simulink model "sf_pole_vault"  (R2025b)
settings: Solver=VariableStepAuto  StartTime=0.0  StopTime=4  MaxStep=.0002  RelTol=1e-3  EnableMultiTasking=on
PreLoadFcn:
  | Params.angle=30;
  | Params.x0=10;
  | Params.y0=3;
  | Params.K=300;
  | Params.mass=100;
  | Params.Pole=4;
  | ang=Params.angle;
  | theta0=ang*pi/180;
  | ltheta0=(Params.x0*sin(theta0)+Params.y0*cos(theta0))/4;
  | r0=Params.y0*sin(theta0)-Params.x0*cos(theta0);
libraries: simulink_extras x3, simulink x1
settings Model: PauseTimes=1.31  Creator=The MathWorks, Inc.  LastModifiedBy=The MathWorks, Inc.
settings SolverCC: AlgebraicLoopSolver=TrustRegion  MaxZcPerStep=1.0
settings DataIOCC: ReturnWorkspaceOutputs=off
settings OptimizationCC: ReuseModelBlockBuffer=off  LifeSpan=inf
settings DebuggingCC: UnconnectedInputMsg=warning  UnconnectedOutputMsg=warning  UnconnectedLineMsg=warning  SFUnexpectedBacktrackingDiag=warning  SFNoUnconditionalDefaultTransitionDiag=warning  SFExecutionAtInitializationDiag=none  ArithmeticOperatorsInVariantConditions=warning
settings ModelReferenceCC: EnableRefExpFcnMdlSchedulingChecks=on
settings SFSimCC: SimUseLocalCustomCode=off  CustomCodeUndefinedFunction=UseInterfaceOnly
settings RTWCC: RTWUseLocalCustomCode=off  GPUComputeCapability=3.5  DLArmComputeVersion=19.05
settings CodeAppCC: StateflowObjectComments=on
settings GRTTargetCC: TargetLangStandard=C89/C90 (ANSI)
settings ConfigComp: CovScope=ReferencedModels  CovIncludeTopModel=off  CovMetricSettings=dw  CovSaveCumulativeToWorkspaceVar=on  CovSaveSingleToWorkspaceVar=on  CovExternalEMLEnable=off

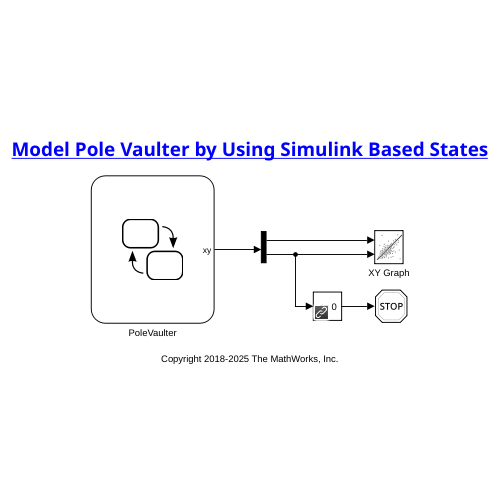
[thumbnail: Simulink's stored preview of the top-level diagram]
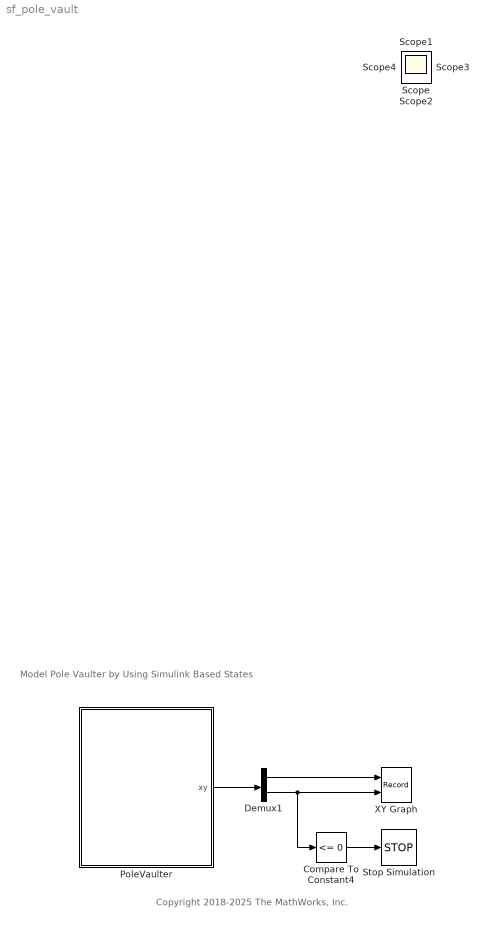
== system sf_pole_vault ==
  note: Copyright 2018-2025 The MathWorks, Inc.
  note: Model Pole Vaulter by Using Simulink Based States
  Compare To Constant4 : simulink/Logic and Bit Operations/Compare To Constant  relop=<=  const=0  OutDataTypeStr=boolean
  Demux1 : Demux  Outputs=2
  PoleVaulter : Stateflow chart  TreatAsAtomicUnit=on
  Stop Simulation : Stop
  XY Graph : Record  NumPorts=2.0  FileSettingsInternal="{\"entries\":[{\"content\":{\"excelSettings\":{\"content\":{},\"type\":\"Streamout.ExcelSettings\"},\"parquetSettings\":{\"content\":{},\"type\":\"Streamout.ParquetSettings\"}},\"type\":\"Streamout.FileSettingStorage\",\"uuid\":\"\"}],\"packageUris\":[\"http:\\/\\/schema.mathworks.com\\/mf0\\/streamout_blocks\\/R2020a\"],\"version\":\"1.0\"}"  FrameSettings=[0, 0]  Layout=[1 1]  SignalsInternal="{\"entries\":[{\"content\":{\"signals\":[{\"content\":{\"blockPath\":[],\"dimensions\":[1],\"domain\":\"\",\"lineColor\":\"#a2142f\",\"plots\":[ 1 ],\"port\":1,\"signalID\":1,\"signalName\":\"XY Graph:1\"},\"type\":\"RecordBlkView.Signal\",\"uuid\":\"\"},{\"content\":{\"blockPath\":[],\"dimensions\":[1],\"domain\":\"\",\"lineColor\":\"#139fff\",\"plots\":[ 1 ],\"port\":2,\"signalID\":2,\"signalName\":\"XY Graph:2\"},\"type\":\"RecordBlkView.Signal\",\"uuid\":\"\"}]},\"type\":\"RecordBlkView.InputSignals\",\"uuid\":\"\"}],\"packageUris\":[\"http:\\/\\/schema.mathworks.com\\/mf0\\/streamout_blocks\\/R2020a\"],\"version\":\"1.0\"}"  VisualizationBindings="{\"xyplotplugin\":{\"info\":[{\"series\":[{\"bindingParametersList\":[{\"parameter\":\"X-Axis\",\"signalID\":1,\"signalName\":\"XY Graph:1\"},{\"parameter\":\"Y-Axis\",\"signalID\":2,\"signalName\":\"XY Graph:2\"}],\"seriesID\":0}],\"subplotID\":1}]}}"  CompatibilityTag=XY  st=-1
  Scope{,1..4} (5 alike) : Scope
      Scope settings: ActiveDisplayYMinimum=-0.125  ActiveDisplayYMaximum=1.125  DataLoggingVariableName=ScopeData2
      Scope1 settings: ActiveDisplayYMinimum=-1  ActiveDisplayYMaximum=1  DataLoggingVariableName=ScopeData3
      Scope2 settings: ActiveDisplayYMinimum=-9.69557  ActiveDisplayYMaximum=6.21487  DataLoggingVariableName=ScopeData4
      Scope3 settings: ActiveDisplayYMinimum=-24.07156  ActiveDisplayYMaximum=216.644  DataLoggingVariableName=ScopeData5
      Scope4 settings: ActiveDisplayYMinimum=-0.125  ActiveDisplayYMaximum=1.125  DataLoggingVariableName=ScopeData6
  wires:
  PoleVaulter/1(xy) -> Demux1/1
  Compare To Constant4/1 -> Stop Simulation/1
  Demux1/1 -> XY Graph/1
  Demux1/2 -> XY Graph/2, Compare To Constant4/1

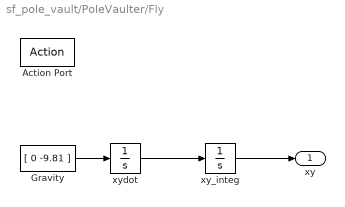
== system sf_pole_vault/PoleVaulter/Fly ==
  Action Port : ActionPort
      settings: CopyFcn=Stateflow.SLINSF.SimulinkMan.removeBlockPreDeleteFcn  PreDeleteFcn=Stateflow.SLINSF.SimulinkMan.unsafePredeleteFcn
  Gravity : Constant  Value=[ 0 -9.81 ]
  xy_integ : Integrator
  xydot : Integrator
  xy : Outport  VectorParamsAs1DForOutWhenUnconnected=off
  wires:
  Gravity/1 -> xydot/1
  xydot/1 -> xy_integ/1
  xy_integ/1 -> xy/1

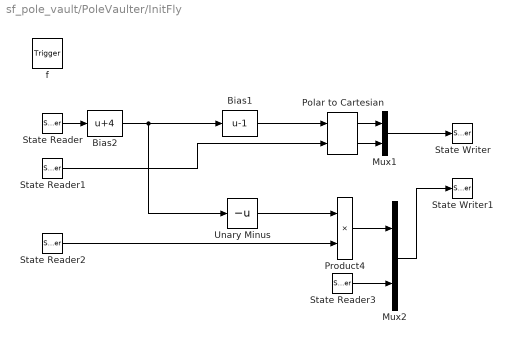
== system sf_pole_vault/PoleVaulter/InitFly ==
  f : TriggerPort  TriggerType=function-call  VariantControl=Variant
      settings: CopyFcn=Stateflow.SLINSF.SimulinkMan.removeBlockPreDeleteFcn  PreDeleteFcn=Stateflow.SLINSF.SimulinkMan.unsafePredeleteFcn
  Bias1 : Bias  Bias=-1  SaturateOnIntegerOverflow=off
  Bias2 : Bias  Bias=4  SaturateOnIntegerOverflow=off
  Mux1 : Mux  Inputs=2
  Mux2 : Mux  Inputs=2
  Polar to Cartesian : simulink_extras/Transformations/Polar to Cartesian
  Product4 : Product
  State Reader : StateReader  StateOwnerBlock=../../Take_off/r  StateName=r
  State Reader1 : StateReader  StateOwnerBlock=../../Take_off/theta  StateName=theta
  State Reader2 : StateReader  StateOwnerBlock=../../Take_off/theta_dot  StateName=theta_dot
  State Reader3 : StateReader  StateOwnerBlock=../../Take_off/r_dot  StateName=rdot
  State Writer : StateWriter  StateOwnerBlock=../../Fly/xy_integ
  State Writer1 : StateWriter  StateOwnerBlock=../../Fly/xydot
  Unary Minus : UnaryMinus
  wires:
  Mux1/1 -> State Writer/1
  Mux2/1 -> State Writer1/1
  Polar to Cartesian/1 -> Mux1/1
  State Reader1/1 -> Polar to Cartesian/2
  State Reader/1 -> Bias2/1
  Bias1/1 -> Polar to Cartesian/1
  Product4/1 -> Mux2/1
  Polar to Cartesian/2 -> Mux1/2
  State Reader2/1 -> Product4/2
  State Reader3/1 -> Mux2/2
  Bias2/1 -> Unary Minus/1, Bias1/1
  Unary Minus/1 -> Product4/1

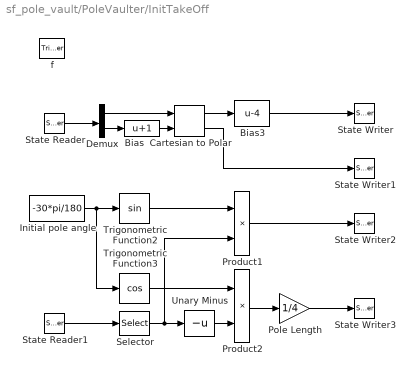
== system sf_pole_vault/PoleVaulter/InitTakeOff ==
  f : TriggerPort  TriggerType=function-call  VariantControl=Variant
      settings: CopyFcn=Stateflow.SLINSF.SimulinkMan.removeBlockPreDeleteFcn  PreDeleteFcn=Stateflow.SLINSF.SimulinkMan.unsafePredeleteFcn
  Bias : Bias  Bias=1  SaturateOnIntegerOverflow=off
  Bias3 : Bias  Bias=-4  SaturateOnIntegerOverflow=off
  Cartesian to Polar : simulink_extras/Transformations/Cartesian to Polar
  Demux : Demux  Outputs=2
  Initial pole angle : Constant  Value=-30*pi/180
  Pole Length : Gain  Gain=1/4
  Product1 : Product
  Product2 : Product
  Selector : Selector  InputPortWidth=2  IndexOptions=Index vector (dialog)  Indices=1  OutputSizes=1
  State Reader : StateReader  StateOwnerBlock=../../Run_up/Position  StateName=p
  State Reader1 : StateReader  StateOwnerBlock=../../Run_up/Velocity  StateName=v
  State Writer : StateWriter  StateOwnerBlock=../../Take_off/r  StateName=r
  State Writer1 : StateWriter  StateOwnerBlock=../../Take_off/theta  StateName=theta
  State Writer2 : StateWriter  StateOwnerBlock=../../Take_off/r_dot  StateName=rdot
  State Writer3 : StateWriter  StateOwnerBlock=../../Take_off/theta_dot  StateName=theta_dot
  Trigonometric Function2 : Trigonometry
  Trigonometric Function3 : Trigonometry  Operator=cos
  Unary Minus : UnaryMinus
  wires:
  Unary Minus/1 -> Product2/2
  Trigonometric Function3/1 -> Product2/1
  Bias3/1 -> State Writer/1
  Selector/1 -> Product1/2, Unary Minus/1
  Trigonometric Function2/1 -> Product1/1
  Product1/1 -> State Writer2/1
  Demux/2 -> Bias/1
  Cartesian to Polar/1 -> Bias3/1
  Bias/1 -> Cartesian to Polar/2
  State Reader/1 -> Demux/1
  Cartesian to Polar/2 -> State Writer1/1
  State Reader1/1 -> Selector/1
  Product2/1 -> Pole Length/1
  Pole Length/1 -> State Writer3/1
  Initial pole angle/1 -> Trigonometric Function3/1, Trigonometric Function2/1
  Demux/1 -> Cartesian to Polar/1

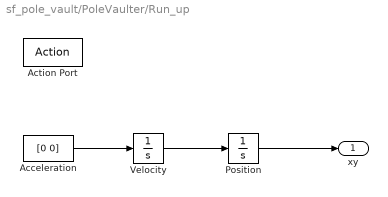
== system sf_pole_vault/PoleVaulter/Run_up ==
  Action Port : ActionPort
      settings: CopyFcn=Stateflow.SLINSF.SimulinkMan.removeBlockPreDeleteFcn  PreDeleteFcn=Stateflow.SLINSF.SimulinkMan.unsafePredeleteFcn
  Acceleration : Constant  Value=[0 0]
  Position : Integrator  InitialCondition=[-10 0.1]  ContinuousStateAttributes='p'
      settings: AttributesFormatString=x0 = %<InitialCondition>
  Velocity : Integrator  InitialCondition=[15 0]  ContinuousStateAttributes='v'
      settings: AttributesFormatString=v0 = %<InitialCondition>
  xy : Outport  VectorParamsAs1DForOutWhenUnconnected=off
  wires:
  Position/1 -> xy/1
  Acceleration/1 -> Velocity/1
  Velocity/1 -> Position/1

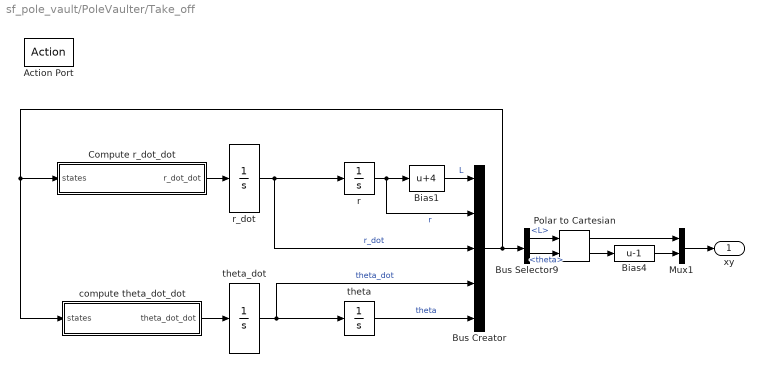
== system sf_pole_vault/PoleVaulter/Take_off ==
  Action Port : ActionPort
      settings: CopyFcn=Stateflow.SLINSF.SimulinkMan.removeBlockPreDeleteFcn  PreDeleteFcn=Stateflow.SLINSF.SimulinkMan.unsafePredeleteFcn
  Bias1 : Bias  Bias=4  SaturateOnIntegerOverflow=off
  Bias4 : Bias  Bias=-1  SaturateOnIntegerOverflow=off
  Bus Creator : BusCreator  Inputs=5
  Bus Selector9 : BusSelector  OutputSignals=L,theta
  Compute r_dot_dot : Subsystem
  Mux1 : Mux  Inputs=2
  Polar to Cartesian : simulink_extras/Transformations/Polar to Cartesian
  compute theta_dot_dot : Subsystem
  r : Integrator  ContinuousStateAttributes='r'
  r_dot : Integrator  InitialCondition=-10*sin(30*pi/180)  ContinuousStateAttributes='rdot'
  theta : Integrator  InitialCondition=theta0  ContinuousStateAttributes='theta'
  theta_dot : Integrator  InitialCondition=10*cos(30*pi/180)/4  ContinuousStateAttributes='theta_dot'
  xy : Outport  VectorParamsAs1DForOutWhenUnconnected=off
  wires:
  r_dot/1 -> Bus Creator/3, r/1  "r_dot"
  r/1 -> Bus Creator/2, Bias1/1  "r"
  theta_dot/1 -> Bus Creator/4, theta/1  "theta_dot"
  Bias1/1 -> Bus Creator/1  "L"
  Bus Creator/1 -> Bus Selector9/1, compute theta_dot_dot/1(states), Compute r_dot_dot/1(states)
  Mux1/1 -> xy/1
  Polar to Cartesian/2 -> Bias4/1
  theta/1 -> Bus Creator/5  "theta"
  Bus Selector9/1 -> Polar to Cartesian/1  "<L>"
  Bus Selector9/2 -> Polar to Cartesian/2  "<theta>"
  Polar to Cartesian/1 -> Mux1/1
  Bias4/1 -> Mux1/2
  Compute r_dot_dot/1(r_dot_dot) -> r_dot/1
  compute theta_dot_dot/1(theta_dot_dot) -> theta_dot/1

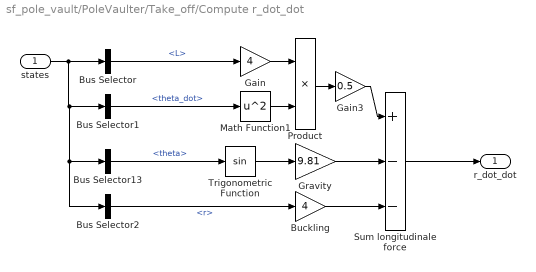
== system sf_pole_vault/PoleVaulter/Take_off/Compute r_dot_dot ==
  states : Inport
  Buckling : Gain  Gain=4
  Bus Selector : BusSelector  OutputSignals=L
  Bus Selector1 : BusSelector  OutputSignals=theta_dot
  Bus Selector13 : BusSelector  OutputSignals=theta
  Bus Selector2 : BusSelector  OutputSignals=r
  Gain : Gain  Gain=4
  Gain3 : Gain  Gain=0.5
  Gravity : Gain  Gain=9.81
  Math Function1 : Math  Operator=square  SignedPower=on
  Product : Product
  Sum longitudinale force : Sum  Inputs=+--
  Trigonometric Function : Trigonometry
  r_dot_dot : Outport  VectorParamsAs1DForOutWhenUnconnected=off
  wires:
  Bus Selector2/1 -> Buckling/1  "<r>"
  Bus Selector/1 -> Gain/1  "<L>"
  Bus Selector1/1 -> Math Function1/1  "<theta_dot>"
  Gain3/1 -> Sum longitudinale force/1
  Gain/1 -> Product/1
  Gravity/1 -> Sum longitudinale force/2
  Buckling/1 -> Sum longitudinale force/3
  Trigonometric Function/1 -> Gravity/1
  Product/1 -> Gain3/1
  Math Function1/1 -> Product/2
  Sum longitudinale force/1 -> r_dot_dot/1
  states/1 -> Bus Selector2/1, Bus Selector13/1, Bus Selector1/1, Bus Selector/1
  Bus Selector13/1 -> Trigonometric Function/1  "<theta>"

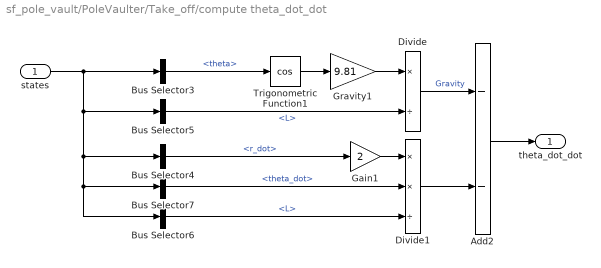
== system sf_pole_vault/PoleVaulter/Take_off/compute theta_dot_dot ==
  states : Inport
  Add2 : Sum  Inputs=--
  Bus Selector3 : BusSelector  OutputSignals=theta
  Bus Selector4 : BusSelector  OutputSignals=r_dot
  Bus Selector5 : BusSelector  OutputSignals=L
  Bus Selector6 : BusSelector  OutputSignals=L
  Bus Selector7 : BusSelector  OutputSignals=theta_dot
  Divide : Product  Inputs=*/
  Divide1 : Product  Inputs=**/
  Gain1 : Gain  Gain=2
  Gravity1 : Gain  Gain=9.81
  Trigonometric Function1 : Trigonometry  Operator=cos
  theta_dot_dot : Outport  VectorParamsAs1DForOutWhenUnconnected=off
  wires:
  Bus Selector3/1 -> Trigonometric Function1/1  "<theta>"
  Bus Selector4/1 -> Gain1/1  "<r_dot>"
  Bus Selector6/1 -> Divide1/3  "<L>"
  Bus Selector5/1 -> Divide/2  "<L>"
  Bus Selector7/1 -> Divide1/2  "<theta_dot>"
  Trigonometric Function1/1 -> Gravity1/1
  Divide1/1 -> Add2/2
  Divide/1 -> Add2/1  "Gravity"
  Gain1/1 -> Divide1/1
  Add2/1 -> theta_dot_dot/1
  states/1 -> Bus Selector5/1, Bus Selector6/1, Bus Selector7/1, Bus Selector4/1, Bus Selector3/1
  Gravity1/1 -> Divide/1

== stateflow chart sf_pole_vault/PoleVaulter ==
  state Run_up
  state InitTakeOff [function]
  state Take_off
  state InitFly [function]
  state Fly
  (default) -> Run_up
  Run_up -> Take_off : [Run_up.p(1) > -4]
      | {InitTakeOff();}
  Take_off -> Fly : [Take_off.theta < pi/2]
      | {InitFly();}
  data: sf_internal_action_state_placeholder_data local double size=1 =0; p local; sf_internal_action_state_placeholder_data local double size=1 =0; theta local; sf_internal_action_state_placeholder_data local double size=1 =0; xy output
